simulink model "VSDk_PMSM_6"  (R2024a)
settings: Solver=VariableStepAuto  StartTime=0.0  StopTime=10.0  RelTol=1e-3
values from neighbouring files (symbols this model uses):
  faif = 0.1351    [init.m]
  Iq_limit = Tn/(1.5*p*faif)*1    (= 90.6192943499)    [init.m]
  Jm = 0.36    [init.m]
  Ki_id_vsd = Rs * wc    (= 61.7197292724)    [init.m]
  Ki_iq_vsd = Rs * wc    (= 61.7197292724)    [init.m]
  Ki_x = Rs * wc_xy    (= 61.7197292724)    [init.m]
  Ki_y = Rs * wc_xy    (= 61.7197292724)    [init.m]
  Kis_vsd = (ws^2 * Jm) / KT    (= 438.324399752)    [init.m]
  Kp_id_vsd = Ld_eff * wc    (= 0.485061905714)    [init.m]
  Kp_iq_vsd = Lq_eff * wc    (= 0.485061905714)    [init.m]
  Kp_x = Lx * wc_xy    (= 0.020106192983)    [init.m]
  Kp_y = Ly * wc_xy    (= 0.020106192983)    [init.m]
  Kps_vsd = (2 * zeta * ws * Jm) / KT    (= 19.7285507573)    [init.m]
  LD = Ld+Ldd    (= 7.72e-05)    [init.m]
  Ld = 40.2e-6    (= 4.02e-05)    [init.m]
  Ldd = 37e-6    (= 3.7e-05)    [init.m]
  Ldz = Ld-Ldd    (= 3.2e-06)    [init.m]
  LQ = Lq+Lqq    (= 7.72e-05)    [init.m]
  Lq = 40.2e-6    (= 4.02e-05)    [init.m]
  Lqq = 37e-6    (= 3.7e-05)    [init.m]
  n = 2000    [init.m]
  p = 4    [init.m]
  Rs = 9.823e-3    (= 0.009823)    [init.m]
  Tn = 734.56/10    (= 73.456)    [init.m]
  Ts = 1/(16e3)    (= 6.25e-05)    [init.m]
  Ts_FEA = 1e-7    (= 1e-07)    [init.m]
  VDC = 1200    [init.m]
  wc_xy = 2 * pi * fc_xy    (= 6283.18530718)    [init.m]
libraries: spsIGBTDiodeLib x24, spsVoltageMeasurementLib x16, spsSeriesRLCBranchLib x12, spsDiodeLib x12, spsOnDelayLib x12, slpidlib x11, simulink x7, spsControlledCurrentSourceLib x6, spsDCVoltageSourceLib x1, spsdq0toAlphaBetaZeroLib x1, spspowerguiLib x1
(part 1 of 3)
settings Model: SimulationMode=accelerator  Creator=Downstream  LastModifiedBy=NitrenePL-SAT
settings DebuggingCC: UnderspecifiedInitializationDetection=Classic  MergeDetectMultiDrivingBlocksExec=none
settings ModelReferenceCC: PropagateSignalLabelsOutOfModel=off

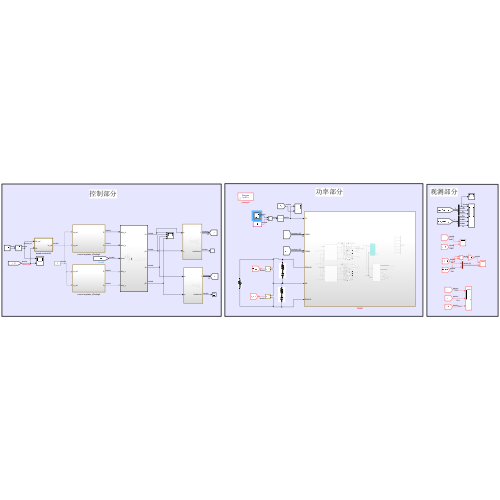
[thumbnail: Simulink's stored preview of the top-level diagram]
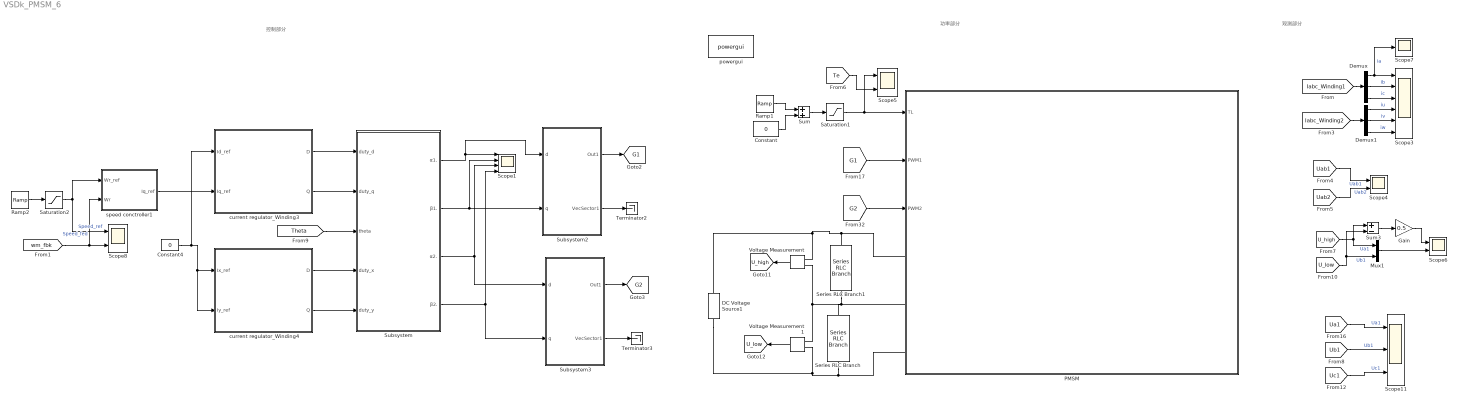
== system VSDk_PMSM_6 ==
  note: 功率部分
  note: 观测部分
  note: 控制部分
  Constant : Constant  Value=0
  Constant4 : Constant  Value=0  SampleTime=-1
  DC Voltage Source1 : spsDCVoltageSourceLib/DC Voltage Source  Amplitude=VDC  Measurements=None
  Demux : Demux  Outputs=3
  Demux1 : Demux  Outputs=3
  Gain : Gain  Gain=0.5
  Mux1 : Mux  Inputs=2
  PMSM : Subsystem
  Ramp1 : simulink/Sources/Ramp  slope=Tn  start=3  InitialOutput=0
  Ramp2 : simulink/Sources/Ramp  slope=n  start=0  InitialOutput=0
  Saturation1 : Saturate  UpperLimit=Tn
  Saturation2 : Saturate  UpperLimit=n
  Scope1 : Scope  NumInputPorts=4
  Scope11 : Scope  NumInputPorts=3
  Scope3 : Scope  NumInputPorts=6
  Scope{4..6,8} (4 alike) : Scope  NumInputPorts=2
  Scope7 : Scope
  Series RLC Branch : spsSeriesRLCBranchLib/Series RLC Branch  LConnTagsString=__new0  RConnTagsString=__new0  BranchType=RC  Resistance=1e-3  Inductance=0  SetiL0=off  InitialCurrent=0  Capacitance=1000e-6  Setx0=off  InitialVoltage=0  Measurements=None
  Series RLC Branch1 : spsSeriesRLCBranchLib/Series RLC Branch  LConnTagsString=__new0  RConnTagsString=__new0  BranchType=RC  Resistance=1e-3  Inductance=0  SetiL0=off  InitialCurrent=0  Capacitance=1000e-6  Setx0=off  InitialVoltage=0  Measurements=None
  Subsystem : Subsystem
  Subsystem2 : Subsystem
  Subsystem3 : Subsystem
  Sum : Sum  OutMax=[Tn]
  Sum3 : Sum  Inputs=+-
  Terminator2 : Terminator
  Terminator3 : Terminator
  Voltage Measurement : spsVoltageMeasurementLib/Voltage Measurement  PhasorSimulation=off  OutputType=Complex  PSBequivalent=0
  Voltage Measurement1 : spsVoltageMeasurementLib/Voltage Measurement  PhasorSimulation=off  OutputType=Complex  PSBequivalent=0
  current regulator_Winding3 : Subsystem
  current regulator_Winding4 : Subsystem
  powergui : spspowerguiLib/powergui  Priority=1  SimulationMode=Discrete  SampleTime=Ts_FEA  frequency=60  Iterations=50  frequencyindice=0  Pbase=100e6  ErrMax=1e-4  UnitsV=kV  UnitsW=MW  buscounter=0  FunctionMessages=off  echomessages=off  EnableUseOfTLC=off  CurrentSourceSwitches=off  DisableSnubberDevices=off  DisableRonSwitches=off  DisableVfSwitches=off  DisplayEquations=off  AutomaticDiscreteSolvers=off  SolverType=Tustin/Backward Euler (TBE)  Interpol=off  ExternalGateDelay=off  methode=off  Ts=100  x0status=blocks  SPID=on  SwTol=0  HookPort=off  NonlinearTolerance=1e-4  nMaxIteration=100  ContinueOnMaxIteration=off  RestoreLinks=warning  ResistiveCurrentMeasurement=off  Frange=[0:2:500]  Ylog=off  Xlog=on  ShowGrid=off  save=off  variable=ZData  structure=IA  ZoomFFT=on  StartTime=0.1927030  cycles=3  DisplayStyle=2  fundamental=816.67  FreqAxis=on  MaxFrequency=816.67*10  frequencyindicesteady=1  RmsSteady=1  display=off
  speed conctroller1 : Subsystem  TreatAsAtomicUnit=on
  tag scope: G1=global, G2=global, U_high=global, U_low=global
  wires:
  [G2] -> PMSM/3(PWM2)
  [G1] -> PMSM/2(PWM1)
  Voltage Measurement1/1 -> [U_low]
  Voltage Measurement/1 -> [U_high]
  Ramp1/1 -> Sum/1
  Constant/1 -> Sum/2
  [Iabc_Winding1] -> Demux/1
  [Iabc_Winding2] -> Demux1/1
  Demux1/3 -> Scope3/6  "iw"
  Demux1/2 -> Scope3/5  "iv"
  Demux1/1 -> Scope3/4  "iu"
  Demux/3 -> Scope3/3  "ic"
  Demux/2 -> Scope3/2  "ib"
  Demux/1 -> Scope7/1, Scope3/1  "ia"
  [Uab1] -> Scope4/1  "Uab1"
  [Uab2] -> Scope4/2  "Uab2"
  Sum/1 -> Saturation1/1
  Saturation1/1 -> PMSM/1(TL), Scope5/1
  [Te] -> Scope5/2
  Constant4/1 -> current regulator_Winding3/1(Id_ref), current regulator_Winding4/2(Iy_ref), current regulator_Winding4/1(Ix_ref)
  Subsystem2/2(VecSector1) -> Terminator2/1
  Subsystem2/1(Out1) -> [G1]
  Ramp2/1 -> Saturation2/1
  Subsystem3/2(VecSector1) -> Terminator3/1
  Saturation2/1 -> speed conctroller1/1(Wr_ref), Scope8/1  "Speed_ref"
  Subsystem3/1(Out1) -> [G2]
  speed conctroller1/1(Iq_ref) -> current regulator_Winding3/2(Iq_ref)
  [Ua1] -> Scope11/1  "Ua1"
  [Ub1] -> Scope11/2  "Ub1"
  [Uc1] -> Scope11/3  "Uc1"
  Sum3/1 -> Gain/1
  [U_high] -> Mux1/1, Sum3/1  "Ua1"
  [U_low] -> Mux1/2, Sum3/2  "Ub1"
  Gain/1 -> Scope6/1
  Mux1/1 -> Scope6/2
  [Theta] -> Subsystem/3(theta)
  current regulator_Winding3/1(D) -> Subsystem/1(duty_d)
  current regulator_Winding3/2(Q) -> Subsystem/2(duty_q)
  current regulator_Winding4/1(D) -> Subsystem/4(duty_x)
  current regulator_Winding4/2(Q) -> Subsystem/5(duty_y)
  Subsystem/1(α1.) -> Subsystem2/1(d), Scope1/1
  Subsystem/4(β2.) -> Subsystem3/2(q), Scope1/4
  Subsystem/2(β1.) -> Subsystem2/2(q), Scope1/2
  Subsystem/3(α2.) -> Scope1/3, Subsystem3/1(d)
  [wm_fbk] -> Scope8/2, speed conctroller1/2(Wr)  "Speed_fed"
  connections:
  Voltage Measurement1/LConn2 -- DC Voltage Source1/LConn1 -- PMSM/LConn3 -- Series RLC Branch/RConn1
  Voltage Measurement/LConn1 -- DC Voltage Source1/RConn1 -- Series RLC Branch1/LConn1 -- PMSM/LConn1
  Voltage Measurement/LConn2 -- Series RLC Branch/LConn1 -- Series RLC Branch1/RConn1 -- PMSM/LConn2 -- Voltage Measurement1/LConn1

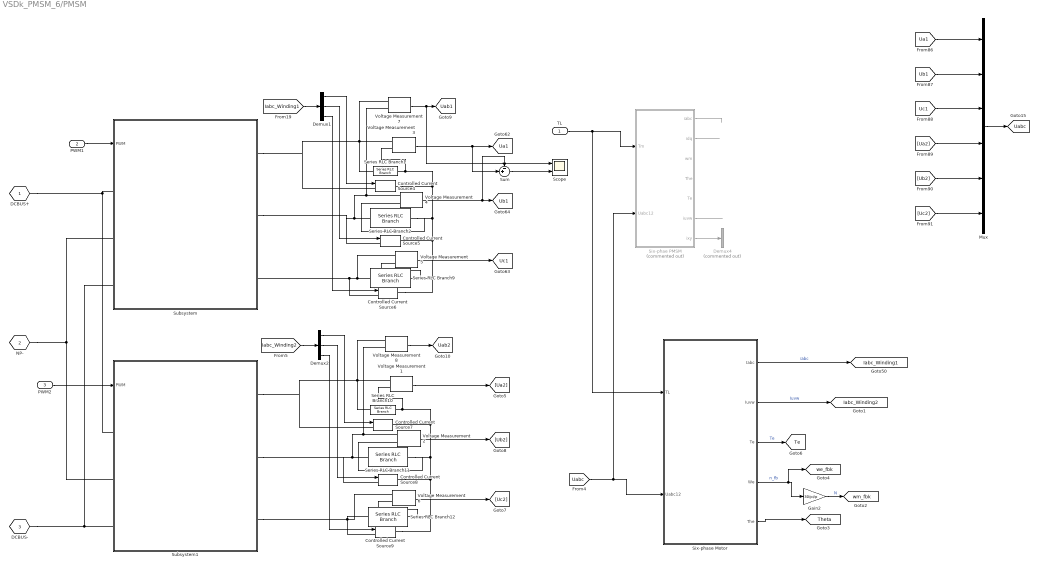
== system VSDk_PMSM_6/PMSM ==
  TL : Inport
  PWM1 : Inport  Port=2
  PWM2 : Inport  Port=3
  Controlled Current Source{4..9} (6 alike) : spsControlledCurrentSourceLib/Controlled Current Source  Initialize=on  Source_Type=AC  Amplitude=0  Phase=0  Frequency=0  Measurements=None
  Demux1 : Demux  Outputs=3
  Demux2 : Demux  Outputs=3
  Demux4 : Demux  Commented=on  Outputs=2
  Gain2 : Gain  Gain=30/pi/p
  Mux : Mux  Inputs=6
  Scope : Scope  NumInputPorts=2
  Series RLC Branch{1..2,9..12} (6 alike) : spsSeriesRLCBranchLib/Series RLC Branch  LConnTagsString=__new0  RConnTagsString=__new0  BranchType=R  Resistance=10^6  Inductance=1e-3  SetiL0=off  InitialCurrent=0  Capacitance=1e-6  Setx0=off  InitialVoltage=0  Measurements=None
  Six-phae PMSM : Subsystem  Commented=on  mask{R=Rs, Ld=LD, Lq=LQ, Lz=Ldz, Flux=faif, J=Jm, F=0, p=p}
      mask prompts: R "R(ohm)"; Ld "Ld(H)"; Lq "Lq(H)"; Lz "Lz(H)"; Flux "Flux(Wb)"; J "J(kg.m^2)"; F "F(N.m.s)"
  Six-phase Motor : Subsystem  mask{Rs=Rs, Ld=Ld, Lq=Lq, Ldd=Ldd, Lqq=Lqq, Flux=faif, B=0, Pn=p, J=Jm}
      mask prompts: Rs "R(ohm)"; Ld "Ld(H)"; Lq "Lq(H)"; Ldd "Ldd(H)"; Lqq "Lqq(H)"; Flux "Flux(wb)"; J "J(kg*m^2)"
      mask DialogControl DescTextVar Prompt: six phase motor
      mask DialogControl Control2 Prompt: Stator Resistance
      mask DialogControl Rs Tooltip: Stator Resistance
      mask DialogControl Control3 Prompt: Stator  d axis Inductance
      mask DialogControl Control4 Prompt: Stator  q axis Inductance
      mask DialogControl Control5 Prompt: Stator  d axis Mutual Inductance
      mask DialogControl Control6 Prompt: Stator  q axis Mutual Inductance
      mask DialogControl Control7 Prompt: Flux linkage
      mask DialogControl Control8 Prompt: damping coefficient
      mask DialogControl Control9 Prompt: motor pole pairs
      mask DialogControl Control10 Prompt: rotational intertia
  Subsystem : Subsystem
  Subsystem1 : Subsystem
  Sum : Sum  Inputs=-+|
  Voltage Measurement{1..8} (8 alike) : spsVoltageMeasurementLib/Voltage Measurement  PhasorSimulation=off  OutputType=Complex  PSBequivalent=0
  DCBUS+ : PMIOPort  Tag=PMCPort  Side=Left
  NP- : PMIOPort  Tag=PMCPort  Port=2  Side=Left
  DCBUS- : PMIOPort  Tag=PMCPort  Port=3  Side=Left
  tag scope: Iabc_Winding1=global, Iabc_Winding2=global, Te=global, Theta=global, Ua1=global, Uab1=global, Uab2=global, Uabc=global, Ub1=global, Uc1=global, we_fbk=global, wm_fbk=global
  wires:
  [Uc2] -> Mux/6
  [Ua2] -> Mux/4
  [Ua1] -> Mux/1
  [Ub1] -> Mux/2
  [Ub2] -> Mux/5
  [Uc1] -> Mux/3
  Mux/1 -> [Uabc]
  Six-phase Motor/4(We) -> Gain2/1, [we_fbk]  "n_fb"
  Six-phase Motor/5(The) -> [Theta]
  Six-phase Motor/3(Te) -> [Te]  "Te"
  PWM1/1 -> Subsystem/1(PWM)
  PWM2/1 -> Subsystem1/1(PWM)
  Demux1/3 -> Controlled Current Source6/1
  Voltage Measurement3/1 -> Sum/2, [Ua1]
  Demux1/2 -> Controlled Current Source5/1
  Voltage Measurement5/1 -> [Uc1]
  Demux1/1 -> Controlled Current Source4/1
  [Iabc_Winding1] -> Demux1/1
  Demux2/2 -> Controlled Current Source8/1
  [Iabc_Winding2] -> Demux2/1
  Demux2/3 -> Controlled Current Source9/1
  Voltage Measurement1/1 -> [Ua2]
  Demux2/1 -> Controlled Current Source7/1
  Voltage Measurement2/1 -> [Ub2]
  Voltage Measurement6/1 -> [Uc2]
  Voltage Measurement7/1 -> Scope/1, [Uab1]
  Voltage Measurement8/1 -> [Uab2]
  TL/1 -> Six-phase Motor/1(TL), Six-phae PMSM/1(Tm)
  Gain2/1 -> [wm_fbk]  "N"
  Six-phae PMSM/7(ixy) -> Demux4/1
  Voltage Measurement4/1 -> Sum/1, [Ub1]
  Sum/1 -> Scope/2
  Six-phase Motor/1(Iabc) -> [Iabc_Winding1]  "iabc"
  Six-phase Motor/2(Iuvw) -> [Iabc_Winding2]  "Iuvw"
  Six-phae PMSM/1(iabc) -> ?
  Six-phae PMSM/2(idq) -> ?
  Six-phae PMSM/6(iuvw) -> ?
  [Uabc] -> Six-phae PMSM/2(Uabc12), Six-phase Motor/2(Uabc12)
  connections:
  DCBUS+/RConn1 -- Subsystem1/LConn1 -- Subsystem/LConn1
  NP-/RConn1 -- Subsystem/LConn2 -- Subsystem1/LConn2
  DCBUS-/RConn1 -- Subsystem1/LConn3 -- Subsystem/LConn3
  Voltage Measurement3/LConn2 -- Series RLC Branch1/LConn1 -- Controlled Current Source4/RConn1 -- Voltage Measurement4/LConn2 -- Series RLC Branch2/LConn1 -- Controlled Current Source5/RConn1 -- Controlled Current Source6/RConn1 -- Series RLC Branch9/LConn1 -- Voltage Measurement5/LConn2
  Voltage Measurement5/LConn1 -- Series RLC Branch9/RConn1 -- Controlled Current Source6/LConn1 -- Subsystem/RConn3
  Voltage Measurement4/LConn1 -- Voltage Measurement7/LConn2 -- Series RLC Branch2/RConn1 -- Subsystem/RConn2 -- Controlled Current Source5/LConn1
  Voltage Measurement3/LConn1 -- Series RLC Branch1/RConn1 -- Voltage Measurement7/LConn1 -- Controlled Current Source4/LConn1 -- Subsystem/RConn1
  Controlled Current Source9/LConn1 -- Subsystem1/RConn3 -- Series RLC Branch12/RConn1 -- Voltage Measurement6/LConn1
  Voltage Measurement1/LConn2 -- Series RLC Branch10/LConn1 -- Controlled Current Source7/RConn1 -- Voltage Measurement2/LConn2 -- Series RLC Branch11/LConn1 -- Controlled Current Source8/RConn1 -- Controlled Current Source9/RConn1 -- Series RLC Branch12/LConn1 -- Voltage Measurement6/LConn2
  Voltage Measurement2/LConn1 -- Voltage Measurement8/LConn2 -- Series RLC Branch11/RConn1 -- Subsystem1/RConn2 -- Controlled Current Source8/LConn1
  Voltage Measurement1/LConn1 -- Voltage Measurement8/LConn1 -- Subsystem1/RConn1 -- Controlled Current Source7/LConn1 -- Series RLC Branch10/RConn1

== system VSDk_PMSM_6/Subsystem ==
  duty_d : Inport
  duty_q : Inport  Port=2
  theta : Inport  Port=3
  duty_x : Inport  Port=4
  duty_y : Inport  Port=5
  Constant2 : Constant  Value=0
  Demux2 : Demux  Outputs=3
  Mux : Mux  Inputs=3
  Mux2 : Mux
  Scope : Scope
  dq0 to Alpha-Beta-Zero : spsdq0toAlphaBetaZeroLib/dq0 to Alpha-Beta-Zero  Alignment=Aligned with phase A axis
  α1 : Fcn  Expr=u(1)+u(3)
  α2 : Fcn  Expr=(sqrt(3)*u(1)+u(2)-sqrt(3)*u(3)+u(4))/2
  β1 : Fcn  Expr=u(2)-u(4)
  β2 : Fcn  Expr=(-u(1)+sqrt(3)*u(2)+u(3)+sqrt(3)*u(4))/2
  α1. : Outport
  β1. : Outport  Port=2
  α2. : Outport  Port=3
  β2. : Outport  Port=4
  wires:
  duty_x/1 -> Mux2/3
  Demux2/1 -> Mux2/1
  Mux/1 -> dq0 to Alpha-Beta-Zero/1
  Constant2/1 -> Mux/3
  Mux2/1 -> Scope/1, β2/1, α2/1, α1/1, β1/1
  duty_y/1 -> Mux2/4
  Demux2/2 -> Mux2/2
  dq0 to Alpha-Beta-Zero/1 -> Demux2/1
  duty_q/1 -> Mux/2
  duty_d/1 -> Mux/1
  theta/1 -> dq0 to Alpha-Beta-Zero/2
  α1/1 -> α1./1
  β1/1 -> β1./1
  α2/1 -> α2./1
  β2/1 -> β2./1

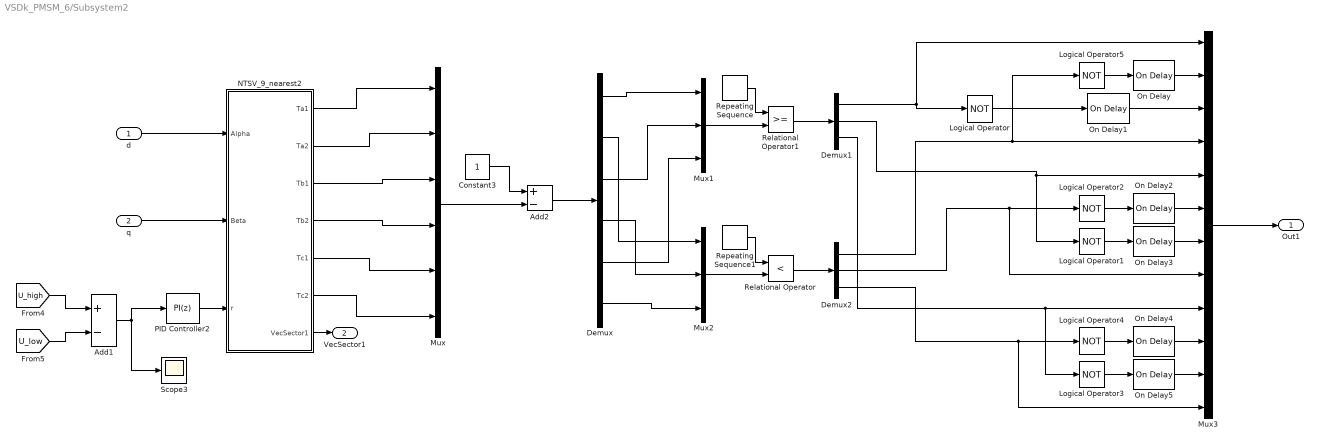
== system VSDk_PMSM_6/Subsystem2 ==
  d : Inport
  q : Inport  Port=2
  Add1 : Sum  Inputs=+-
  Add2 : Sum  Inputs=+-
  Constant3 : Constant
  Demux : Demux  Outputs=6
  Demux1 : Demux  Outputs=3
  Demux2 : Demux  Outputs=3
  Logical Operator{,1..5} (6 alike) : Logic  Operator=NOT  AllPortsSameDT=off  OutDataTypeStr=boolean
  Mux : Mux  Inputs=6
  Mux1 : Mux  Inputs=3
  Mux2 : Mux  Inputs=3
  Mux3 : Mux  Inputs=12
  NTSV_9_nearest2 : MATLAB Function  TreatAsAtomicUnit=on
  On Delay{,1..5} (6 alike) : spsOnDelayLib/On Delay  DelayType=On delay  delay=Ts_Dead  ic=0  Ts=0
  PID Controller2 : slpidlib/PID Controller  Controller=PI  Form=Parallel  TimeDomain=Discrete-time  UseExternalTs=off  SampleTime=Ts  IntegratorMethod=Forward Euler  FilterMethod=Forward Euler  ControllerParametersSource=internal  P=0.005  I=0.05  UseKiTs=off  D=0  UseExternalDerivativeSource=off  N=100  UseFilter=on  TunerSelectOption=Transfer Function Based (PID Tuner App)  InitialConditionSource=internal  InitialConditionForIntegrator=0  InitialConditionForFilter=0  DifferentiatorICPrevScaledInput=0  ExternalReset=none  TrackingMode=off  Kt=1  LimitOutput=off  SatLimitsSource=internal  UpperSaturationLimit=inf  LowerSaturationLimit=-inf  LinearizeAsGain=on  AntiWindupMode=none  Kb=1  LimitIntegrator=off  UpperIntegratorSaturationLimit=inf  LowerIntegratorSaturationLimit=-inf  POutMin=[]  POutMax=[]  IOutMin=[]  IOutMax=[]  DOutMin=[]  DOutMax=[]  NOutMin=[]  NOutMax=[]  SumOutMin=[]  SumOutMax=[]  SaturationOutMin=[]  SaturationOutMax=[]  PParamMin=[]  PParamMax=[]  IParamMin=[]  IParamMax=[]  DParamMin=[]  DParamMax=[]  NParamMin=[]  NParamMax=[]  KbParamMin=[]  KbParamMax=[]  KtParamMin=[]  KtParamMax=[]  KbOutMin=[]  KbOutMax=[]  KtOutMin=[]  KtOutMax=[]  IntegratorOutMin=[]  IntegratorOutMax=[]  FilterOutMin=[]  FilterOutMax=[]  SumI1OutMin=[]  SumI1OutMax=[]  SumI2OutMin=[]  SumI2OutMax=[]  SumI3OutMin=[]  SumI3OutMax=[]  SumI4OutMin=[]  SumI4OutMax=[]  SumDOutMin=[]  SumDOutMax=[]  DifferentiatorOutMin=[]  DifferentiatorOutMax=[]  FilterDiffOutCoefMin=[]  FilterDiffOutCoefMax=[]  ReciprocalOutMin=[]  ReciprocalOutMax=[]  SumDenOutMin=[]  SumDenOutMax=[]  SumNumOutMin=[]  SumNumOutMax=[]  DivideOutMin=[]  DivideOutMax=[]  UdiffTsProdOutMin=[]  UdiffTsProdOutMax=[]  NTsProdOutMin=[]  NTsProdOutMax=[]  UintegralTsProdOutMin=[]  UintegralTsProdOutMax=[]  UngainTsProdOutMin=[]  UngainTsProdOutMax=[]  ClampingZeroOutDataTypeStr=Inherit: Inherit via back propagation  ClampingZeroOutMin=[]  ClampingZeroOutMax=[]  FilterDenConstantOutDataTypeStr=Inherit: Inherit via back propagation  FilterDenConstantOutMin=[]  FilterDenConstantOutMax=[]  PCopyOutDataTypeStr=Inherit: Inherit via back propagation  PCopyOutMin=[]  PCopyOutMax=[]  NCopyOutDataTypeStr=Inherit: Inherit via back propagation  NCopyOutMin=[]  NCopyOutMax=[]  IntegratorContinuousStateAttributes=''  IntegratorStateMustResolveToSignalObject=off  IntegratorRTWStateStorageClass=Auto  FilterContinuousStateAttributes=''  FilterStateMustResolveToSignalObject=off  FilterRTWStateStorageClass=Auto  ParallelPVariant=InternalParameters  IdealPVariant=Disabled  IVariant=InternalParameters  DVariant=Disabled  IntegratorVariant=Discrete  SatVariant=Disabled  AWVariant=Passthrough  PCopyVariant=Disabled  TRVariant=Disabled  FdbkBlocksVariant=Forward  IdealPFdbkVariant=Disabled  SatFdbkVariant=Disabled  DerivativeFilterVariant=Disabled  NVariant=Disabled  NCopyVariant=Disabled_SignalSpec  FilterICVariant=Disabled  IntegratorICVariant=InternalICs  ExternalResetVariant=Disabled  TRSumVariant=Passthrough  SumFdbkVariant=Disabled  SumVariant=Sum_PI  TsampFilterVariant=InternalTs  TsampNgainVariant=Passthrough  TsampIntegralVariant=Disabled_SignalSpec  ExternalSaturationOutDataTypeStr=Inherit: Same as second input  DerivativeSourceVariant=Disabled
  Relational Operator : RelationalOperator  Operator=<  OutDataTypeStr=boolean  RndMeth=Simplest  InputSameDT=off
  Relational Operator1 : RelationalOperator  OutDataTypeStr=boolean  RndMeth=Simplest  InputSameDT=off
  Repeating Sequence : simulink/Sources/Repeating Sequence  rep_seq_t=[0 Ts/2 Ts]  rep_seq_y=[0 1 0]
  Repeating Sequence1 : simulink/Sources/Repeating Sequence  rep_seq_t=[0 Ts/2 Ts]  rep_seq_y=[0 1 0]
  Scope3 : Scope
  Out1 : Outport
  VecSector1 : Outport  Port=2
  wires:
  NTSV_9_nearest2/7(VecSector1) -> VecSector1/1
  Demux/1 -> Mux1/1
  Demux2/3 -> Logical Operator4/1, Mux3/12
  Logical Operator4/1 -> On Delay4/1
  Demux/5 -> Mux1/3
  Logical Operator2/1 -> On Delay2/1
  Demux1/1 -> Logical Operator/1, Mux3/1
  Add1/1 -> Scope3/1, PID Controller2/1
  Constant3/1 -> Add2/1
  Demux2/2 -> Mux3/8, Logical Operator2/1
  Demux2/1 -> Logical Operator5/1, Mux3/4
  On Delay1/1 -> Mux3/3
  NTSV_9_nearest2/2(Ta2) -> Mux/2
  On Delay3/1 -> Mux3/7
  Logical Operator5/1 -> On Delay/1
  Relational Operator1/1 -> Demux1/1
  Mux/1 -> Add2/2
  Repeating Sequence1/1 -> Relational Operator/1
  NTSV_9_nearest2/6(Tc2) -> Mux/6
  Demux/2 -> Mux2/1
  Mux1/1 -> Relational Operator1/2
  Mux2/1 -> Relational Operator/2
  PID Controller2/1 -> NTSV_9_nearest2/3(r)
  Add2/1 -> Demux/1
  On Delay/1 -> Mux3/2
  Relational Operator/1 -> Demux2/1
  NTSV_9_nearest2/1(Ta1) -> Mux/1
  [U_low] -> Add1/2
  NTSV_9_nearest2/4(Tb2) -> Mux/4
  Demux/6 -> Mux2/3
  Demux1/3 -> Logical Operator3/1, Mux3/9
  q/1 -> NTSV_9_nearest2/2(Beta)
  On Delay2/1 -> Mux3/6
  [U_high] -> Add1/1
  On Delay5/1 -> Mux3/11
  NTSV_9_nearest2/5(Tc1) -> Mux/5
  Demux1/2 -> Logical Operator1/1, Mux3/5
  d/1 -> NTSV_9_nearest2/1(Alpha)
  Logical Operator3/1 -> On Delay5/1
  On Delay4/1 -> Mux3/10
  Mux3/1 -> Out1/1
  NTSV_9_nearest2/3(Tb1) -> Mux/3
  Logical Operator/1 -> On Delay1/1
  Logical Operator1/1 -> On Delay3/1
  Repeating Sequence/1 -> Relational Operator1/1
  Demux/4 -> Mux2/2
  Demux/3 -> Mux1/2

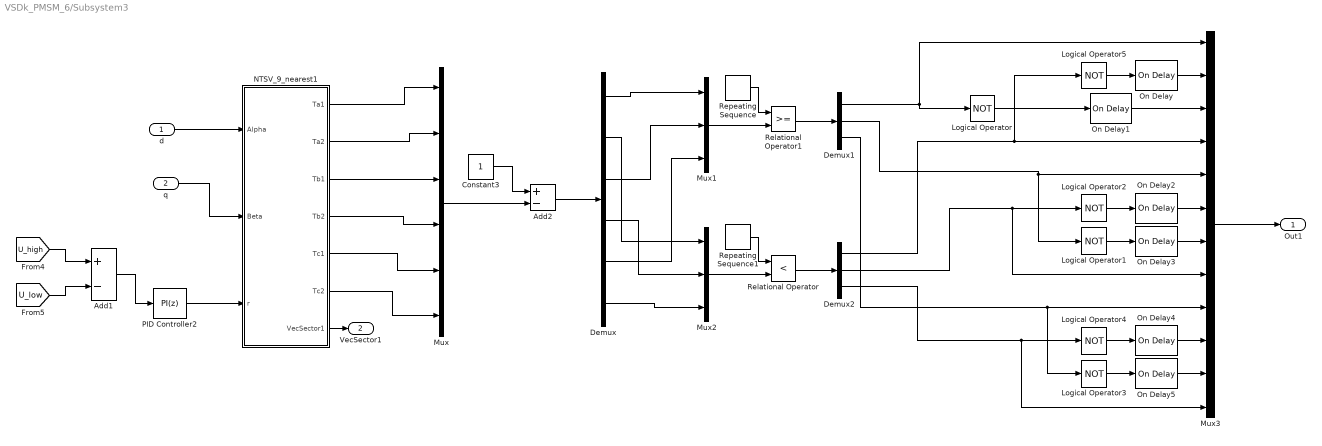
== system VSDk_PMSM_6/Subsystem3 ==
  d : Inport
  q : Inport  Port=2
  Add1 : Sum  Inputs=+-
  Add2 : Sum  Inputs=+-
  Constant3 : Constant
  Demux : Demux  Outputs=6
  Demux1 : Demux  Outputs=3
  Demux2 : Demux  Outputs=3
  Logical Operator{,1..5} (6 alike) : Logic  Operator=NOT  AllPortsSameDT=off  OutDataTypeStr=boolean
  Mux : Mux  Inputs=6
  Mux1 : Mux  Inputs=3
  Mux2 : Mux  Inputs=3
  Mux3 : Mux  Inputs=12
  NTSV_9_nearest1 : MATLAB Function  TreatAsAtomicUnit=on
  On Delay{,1..5} (6 alike) : spsOnDelayLib/On Delay  DelayType=On delay  delay=Ts_Dead  ic=0  Ts=0
  PID Controller2 : slpidlib/PID Controller  Controller=PI  Form=Parallel  TimeDomain=Discrete-time  UseExternalTs=off  SampleTime=Ts  IntegratorMethod=Forward Euler  FilterMethod=Forward Euler  ControllerParametersSource=internal  P=0.005  I=0.05  UseKiTs=off  D=0  UseExternalDerivativeSource=off  N=100  UseFilter=on  TunerSelectOption=Transfer Function Based (PID Tuner App)  InitialConditionSource=internal  InitialConditionForIntegrator=0  InitialConditionForFilter=0  DifferentiatorICPrevScaledInput=0  ExternalReset=none  TrackingMode=off  Kt=1  LimitOutput=off  SatLimitsSource=internal  UpperSaturationLimit=inf  LowerSaturationLimit=-inf  LinearizeAsGain=on  AntiWindupMode=none  Kb=1  LimitIntegrator=off  UpperIntegratorSaturationLimit=inf  LowerIntegratorSaturationLimit=-inf  POutMin=[]  POutMax=[]  IOutMin=[]  IOutMax=[]  DOutMin=[]  DOutMax=[]  NOutMin=[]  NOutMax=[]  SumOutMin=[]  SumOutMax=[]  SaturationOutMin=[]  SaturationOutMax=[]  PParamMin=[]  PParamMax=[]  IParamMin=[]  IParamMax=[]  DParamMin=[]  DParamMax=[]  NParamMin=[]  NParamMax=[]  KbParamMin=[]  KbParamMax=[]  KtParamMin=[]  KtParamMax=[]  KbOutMin=[]  KbOutMax=[]  KtOutMin=[]  KtOutMax=[]  IntegratorOutMin=[]  IntegratorOutMax=[]  FilterOutMin=[]  FilterOutMax=[]  SumI1OutMin=[]  SumI1OutMax=[]  SumI2OutMin=[]  SumI2OutMax=[]  SumI3OutMin=[]  SumI3OutMax=[]  SumI4OutMin=[]  SumI4OutMax=[]  SumDOutMin=[]  SumDOutMax=[]  DifferentiatorOutMin=[]  DifferentiatorOutMax=[]  FilterDiffOutCoefMin=[]  FilterDiffOutCoefMax=[]  ReciprocalOutMin=[]  ReciprocalOutMax=[]  SumDenOutMin=[]  SumDenOutMax=[]  SumNumOutMin=[]  SumNumOutMax=[]  DivideOutMin=[]  DivideOutMax=[]  UdiffTsProdOutMin=[]  UdiffTsProdOutMax=[]  NTsProdOutMin=[]  NTsProdOutMax=[]  UintegralTsProdOutMin=[]  UintegralTsProdOutMax=[]  UngainTsProdOutMin=[]  UngainTsProdOutMax=[]  ClampingZeroOutDataTypeStr=Inherit: Inherit via back propagation  ClampingZeroOutMin=[]  ClampingZeroOutMax=[]  FilterDenConstantOutDataTypeStr=Inherit: Inherit via back propagation  FilterDenConstantOutMin=[]  FilterDenConstantOutMax=[]  PCopyOutDataTypeStr=Inherit: Inherit via back propagation  PCopyOutMin=[]  PCopyOutMax=[]  NCopyOutDataTypeStr=Inherit: Inherit via back propagation  NCopyOutMin=[]  NCopyOutMax=[]  IntegratorContinuousStateAttributes=''  IntegratorStateMustResolveToSignalObject=off  IntegratorRTWStateStorageClass=Auto  FilterContinuousStateAttributes=''  FilterStateMustResolveToSignalObject=off  FilterRTWStateStorageClass=Auto  ParallelPVariant=InternalParameters  IdealPVariant=Disabled  IVariant=InternalParameters  DVariant=Disabled  IntegratorVariant=Discrete  SatVariant=Disabled  AWVariant=Passthrough  PCopyVariant=Disabled  TRVariant=Disabled  FdbkBlocksVariant=Forward  IdealPFdbkVariant=Disabled  SatFdbkVariant=Disabled  DerivativeFilterVariant=Disabled  NVariant=Disabled  NCopyVariant=Disabled_SignalSpec  FilterICVariant=Disabled  IntegratorICVariant=InternalICs  ExternalResetVariant=Disabled  TRSumVariant=Passthrough  SumFdbkVariant=Disabled  SumVariant=Sum_PI  TsampFilterVariant=InternalTs  TsampNgainVariant=Passthrough  TsampIntegralVariant=Disabled_SignalSpec  ExternalSaturationOutDataTypeStr=Inherit: Same as second input  DerivativeSourceVariant=Disabled
  Relational Operator : RelationalOperator  Operator=<  OutDataTypeStr=boolean  RndMeth=Simplest  InputSameDT=off
  Relational Operator1 : RelationalOperator  OutDataTypeStr=boolean  RndMeth=Simplest  InputSameDT=off
  Repeating Sequence : simulink/Sources/Repeating Sequence  rep_seq_t=[0 Ts/2 Ts]  rep_seq_y=[0 1 0]
  Repeating Sequence1 : simulink/Sources/Repeating Sequence  rep_seq_t=[0 Ts/2 Ts]  rep_seq_y=[0 1 0]
  Out1 : Outport
  VecSector1 : Outport  Port=2
  wires:
  NTSV_9_nearest1/7(VecSector1) -> VecSector1/1
  Demux/1 -> Mux1/1
  Demux2/3 -> Logical Operator4/1, Mux3/12
  Logical Operator4/1 -> On Delay4/1
  Demux/5 -> Mux1/3
  Logical Operator2/1 -> On Delay2/1
  Demux1/1 -> Logical Operator/1, Mux3/1
  Add1/1 -> PID Controller2/1
  Constant3/1 -> Add2/1
  Demux2/2 -> Mux3/8, Logical Operator2/1
  Demux2/1 -> Logical Operator5/1, Mux3/4
  On Delay1/1 -> Mux3/3
  NTSV_9_nearest1/2(Ta2) -> Mux/2
  On Delay3/1 -> Mux3/7
  Logical Operator5/1 -> On Delay/1
  Relational Operator1/1 -> Demux1/1
  Mux/1 -> Add2/2
  Repeating Sequence1/1 -> Relational Operator/1
  NTSV_9_nearest1/6(Tc2) -> Mux/6
  Demux/2 -> Mux2/1
  Mux1/1 -> Relational Operator1/2
  Mux2/1 -> Relational Operator/2
  PID Controller2/1 -> NTSV_9_nearest1/3(r)
  Add2/1 -> Demux/1
  On Delay/1 -> Mux3/2
  Relational Operator/1 -> Demux2/1
  NTSV_9_nearest1/1(Ta1) -> Mux/1
  [U_low] -> Add1/2
  NTSV_9_nearest1/4(Tb2) -> Mux/4
  Demux/6 -> Mux2/3
  Demux1/3 -> Logical Operator3/1, Mux3/9
  q/1 -> NTSV_9_nearest1/2(Beta)
  On Delay2/1 -> Mux3/6
  [U_high] -> Add1/1
  On Delay5/1 -> Mux3/11
  NTSV_9_nearest1/5(Tc1) -> Mux/5
  Demux1/2 -> Logical Operator1/1, Mux3/5
  d/1 -> NTSV_9_nearest1/1(Alpha)
  Logical Operator3/1 -> On Delay5/1
  On Delay4/1 -> Mux3/10
  Mux3/1 -> Out1/1
  NTSV_9_nearest1/3(Tb1) -> Mux/3
  Logical Operator/1 -> On Delay1/1
  Logical Operator1/1 -> On Delay3/1
  Repeating Sequence/1 -> Relational Operator1/1
  Demux/4 -> Mux2/2
  Demux/3 -> Mux1/2

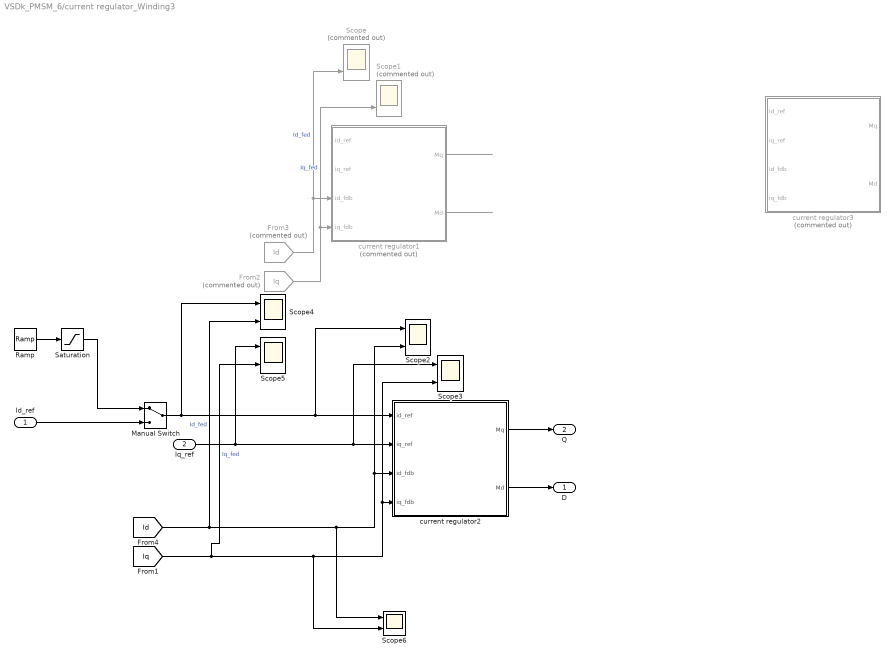
== system VSDk_PMSM_6/current regulator_Winding3 ==
  Id_ref : Inport
  Iq_ref : Inport  Port=2
  From2 : From  Commented=on  GotoTag=Iq  TagVisibility=global
  From3 : From  Commented=on  GotoTag=Id  TagVisibility=global
  Manual Switch : ManualSwitch
  Ramp : simulink/Sources/Ramp  slope=100  start=1.2  InitialOutput=0
  Saturation : Saturate  UpperLimit=200
  Scope : Scope  Commented=on  NumInputPorts=2
  Scope1 : Scope  Commented=on  NumInputPorts=2
  Scope{2..6} (5 alike) : Scope  NumInputPorts=2
  current regulator1 : Subsystem  Commented=on
  current regulator2 : Subsystem
  current regulator3 : Subsystem  Commented=on
  D : Outport  VectorParamsAs1DForOutWhenUnconnected=off
  Q : Outport  Port=2  VectorParamsAs1DForOutWhenUnconnected=off
  wires:
  current regulator1/1(Mq) -> ?
  ? -> Scope/1, current regulator1/1(id_ref)
  current regulator1/2(Md) -> ?
  ? -> Scope1/1, current regulator1/2(iq_ref)
  From3/1 -> Scope/2, current regulator1/3(id_fdb)  "Id_fed"
  From2/1 -> Scope1/2, current regulator1/4(iq_fdb)  "Iq_fed"
  [Iq] -> Scope6/2, Scope3/2, current regulator2/4(iq_fdb), Scope5/2  "Iq_fed"
  [Id] -> Scope6/1, Scope2/2, current regulator2/3(id_fdb), Scope4/2  "Id_fed"
  current regulator2/1(Mq) -> Q/1
  current regulator2/2(Md) -> D/1
  Iq_ref/1 -> Scope3/1, current regulator2/2(iq_ref), Scope5/1
  Ramp/1 -> Saturation/1
  Id_ref/1 -> Manual Switch/2
  Manual Switch/1 -> Scope4/1, Scope2/1, current regulator2/1(id_ref)
  Saturation/1 -> Manual Switch/1

== system VSDk_PMSM_6/current regulator_Winding4 ==
  Ix_ref : Inport
  Iy_ref : Inport  Port=2
  Scope{,1,4..6} (5 alike) : Scope  NumInputPorts=2
  current regulator3 : Subsystem
  D : Outport  VectorParamsAs1DForOutWhenUnconnected=off
  Q : Outport  Port=2  VectorParamsAs1DForOutWhenUnconnected=off
  wires:
  [Iy] -> Scope/2, current regulator3/4(iy_fdb), Scope5/2, Scope6/2  "Iy_fed"
  [Ix] -> Scope/1, current regulator3/3(ix_fdb), Scope4/2, Scope1/2  "Ix_fed"
  Ix_ref/1 -> Scope1/1, current regulator3/1(ix_ref), Scope4/1  "id_fbk"
  Iy_ref/1 -> Scope6/1, current regulator3/2(iy_ref), Scope5/1
  current regulator3/1(My) -> Q/1
  current regulator3/2(Mx) -> D/1

== system VSDk_PMSM_6/speed conctroller1 ==
  Wr_ref : Inport
  Wr : Inport  Port=2
  Add : Sum  Inputs=+-
  PID Controller1 : slpidlib/PID Controller  Controller=PI  Form=Parallel  TimeDomain=Discrete-time  UseExternalTs=off  SampleTime=Ts  IntegratorMethod=Forward Euler  FilterMethod=Forward Euler  ControllerParametersSource=internal  P=Kps_vsd  I=Kis_vsd  UseKiTs=off  D=0  UseExternalDerivativeSource=off  N=100  UseFilter=on  TunerSelectOption=Transfer Function Based (PID Tuner App)  InitialConditionSource=internal  InitialConditionForIntegrator=0  InitialConditionForFilter=0  DifferentiatorICPrevScaledInput=0  ExternalReset=none  TrackingMode=off  Kt=1  LimitOutput=on  SatLimitsSource=internal  UpperSaturationLimit=Iq_limit  LowerSaturationLimit=-Iq_limit  LinearizeAsGain=off  AntiWindupMode=none  Kb=1  LimitIntegrator=off  UpperIntegratorSaturationLimit=inf  LowerIntegratorSaturationLimit=-inf  POutMin=[]  POutMax=[]  IOutMin=[]  IOutMax=[]  DOutMin=[]  DOutMax=[]  NOutMin=[]  NOutMax=[]  SumOutMin=[]  SumOutMax=[]  SaturationOutMin=[]  SaturationOutMax=[]  PParamMin=[]  PParamMax=[]  IParamMin=[]  IParamMax=[]  DParamMin=[]  DParamMax=[]  NParamMin=[]  NParamMax=[]  KbParamMin=[]  KbParamMax=[]  KtParamMin=[]  KtParamMax=[]  KbOutMin=[]  KbOutMax=[]  KtOutMin=[]  KtOutMax=[]  IntegratorOutMin=[]  IntegratorOutMax=[]  FilterOutMin=[]  FilterOutMax=[]  SumI1OutMin=[]  SumI1OutMax=[]  SumI2OutMin=[]  SumI2OutMax=[]  SumI3OutMin=[]  SumI3OutMax=[]  SumI4OutMin=[]  SumI4OutMax=[]  SumDOutMin=[]  SumDOutMax=[]  DifferentiatorOutMin=[]  DifferentiatorOutMax=[]  FilterDiffOutCoefMin=[]  FilterDiffOutCoefMax=[]  ReciprocalOutMin=[]  ReciprocalOutMax=[]  SumDenOutMin=[]  SumDenOutMax=[]  SumNumOutMin=[]  SumNumOutMax=[]  DivideOutMin=[]  DivideOutMax=[]  UdiffTsProdOutMin=[]  UdiffTsProdOutMax=[]  NTsProdOutMin=[]  NTsProdOutMax=[]  UintegralTsProdOutMin=[]  UintegralTsProdOutMax=[]  UngainTsProdOutMin=[]  UngainTsProdOutMax=[]  ClampingZeroOutDataTypeStr=Inherit: Inherit via back propagation  ClampingZeroOutMin=[]  ClampingZeroOutMax=[]  FilterDenConstantOutDataTypeStr=Inherit: Inherit via back propagation  FilterDenConstantOutMin=[]  FilterDenConstantOutMax=[]  PCopyOutDataTypeStr=Inherit: Inherit via back propagation  PCopyOutMin=[]  PCopyOutMax=[]  NCopyOutDataTypeStr=Inherit: Inherit via back propagation  NCopyOutMin=[]  NCopyOutMax=[]  IntegratorContinuousStateAttributes=''  IntegratorStateMustResolveToSignalObject=off  IntegratorRTWStateStorageClass=Auto  FilterContinuousStateAttributes=''  FilterStateMustResolveToSignalObject=off  FilterRTWStateStorageClass=Auto  ParallelPVariant=InternalParameters  IdealPVariant=Disabled  IVariant=InternalParameters  DVariant=Disabled  IntegratorVariant=Discrete  SatVariant=Enabled  AWVariant=Passthrough  PCopyVariant=Disabled  TRVariant=Disabled  FdbkBlocksVariant=Forward  IdealPFdbkVariant=Disabled  SatFdbkVariant=Disabled  DerivativeFilterVariant=Disabled  NVariant=Disabled  NCopyVariant=Disabled_SignalSpec  FilterICVariant=Disabled  IntegratorICVariant=InternalICs  ExternalResetVariant=Disabled  TRSumVariant=Passthrough  SumFdbkVariant=Disabled  SumVariant=Sum_PI  TsampFilterVariant=InternalTs  TsampNgainVariant=Passthrough  TsampIntegralVariant=Disabled_SignalSpec  ExternalSaturationOutDataTypeStr=Inherit: Same as second input  DerivativeSourceVariant=Disabled
  Scope1 : Scope
  Iq_ref : Outport  VectorParamsAs1DForOutWhenUnconnected=off
  wires:
  Add/1 -> PID Controller1/1
  Wr/1 -> Add/2
  PID Controller1/1 -> Iq_ref/1
  Wr_ref/1 -> Scope1/1, Add/1

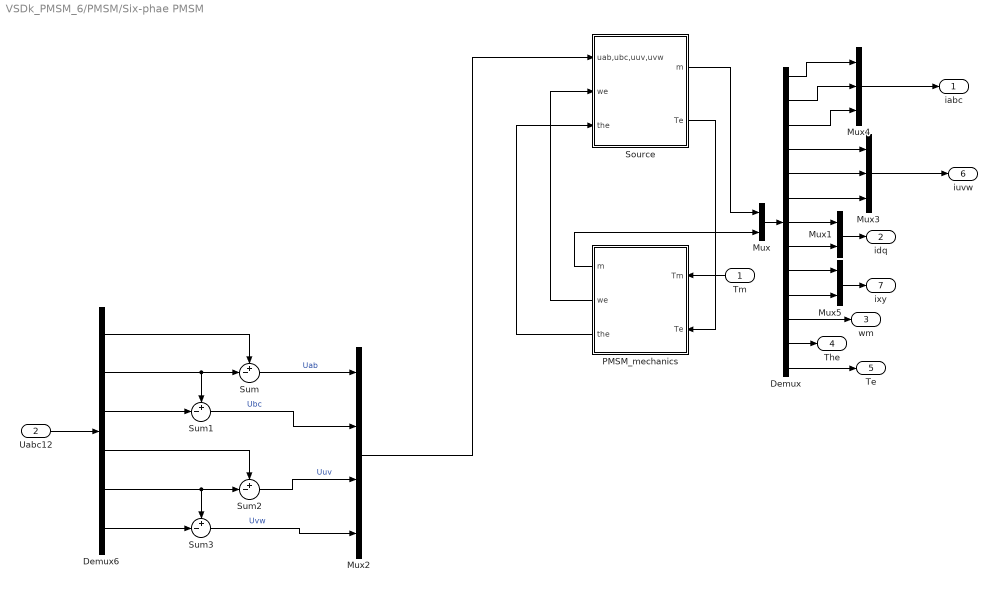
== system VSDk_PMSM_6/PMSM/Six-phae PMSM ==
  Tm : Inport
  Uabc12 : Inport  Port=2
  Demux : Demux  Outputs=13
  Demux6 : Demux  Outputs=6
  Mux : Mux  Inputs=2
  Mux1 : Mux  Inputs=2
  Mux2 : Mux
  Mux3 : Mux  Inputs=3
  Mux4 : Mux  Inputs=3
  Mux5 : Mux  Inputs=2
  PMSM_mechanics : Subsystem
  Source : Subsystem
  Sum{,1..3} (4 alike) : Sum  Inputs=+-|
  iabc : Outport
  idq : Outport  Port=2
  wm : Outport  Port=3
  The : Outport  Port=4
  Te : Outport  Port=5
  iuvw : Outport  Port=6
  ixy : Outport  Port=7
  wires:
  Tm/1 -> PMSM_mechanics/1(Tm)
  Source/2(Te) -> PMSM_mechanics/2(Te)
  PMSM_mechanics/2(we) -> Source/2(we)
  PMSM_mechanics/3(the) -> Source/3(the)
  PMSM_mechanics/1(m) -> Mux/2
  Source/1(m) -> Mux/1
  Mux/1 -> Demux/1
  Mux4/1 -> iabc/1
  Mux1/1 -> idq/1
  Demux/12 -> The/1
  Demux/13 -> Te/1
  Demux/5 -> Mux3/2
  Demux/2 -> Mux4/2
  Demux/3 -> Mux4/3
  Demux/6 -> Mux3/3
  Demux/4 -> Mux3/1
  Demux/1 -> Mux4/1
  Demux/7 -> Mux1/1
  Demux/8 -> Mux1/2
  Demux/9 -> Mux5/1
  Demux/10 -> Mux5/2
  Demux/11 -> wm/1
  Uabc12/1 -> Demux6/1
  Demux6/2 -> Sum1/1, Sum/2
  Demux6/1 -> Sum/1
  Demux6/3 -> Sum1/2
  Sum/1 -> Mux2/1  "Uab"
  Sum1/1 -> Mux2/2  "Ubc"
  Sum3/1 -> Mux2/4  "Uvw"
  Sum2/1 -> Mux2/3  "Uuv"
  Demux6/5 -> Sum3/1, Sum2/2
  Demux6/4 -> Sum2/1
  Demux6/6 -> Sum3/2
  Mux2/1 -> Source/1(uab,ubc,uuv,uvw)
  Mux3/1 -> iuvw/1
  Mux5/1 -> ixy/1

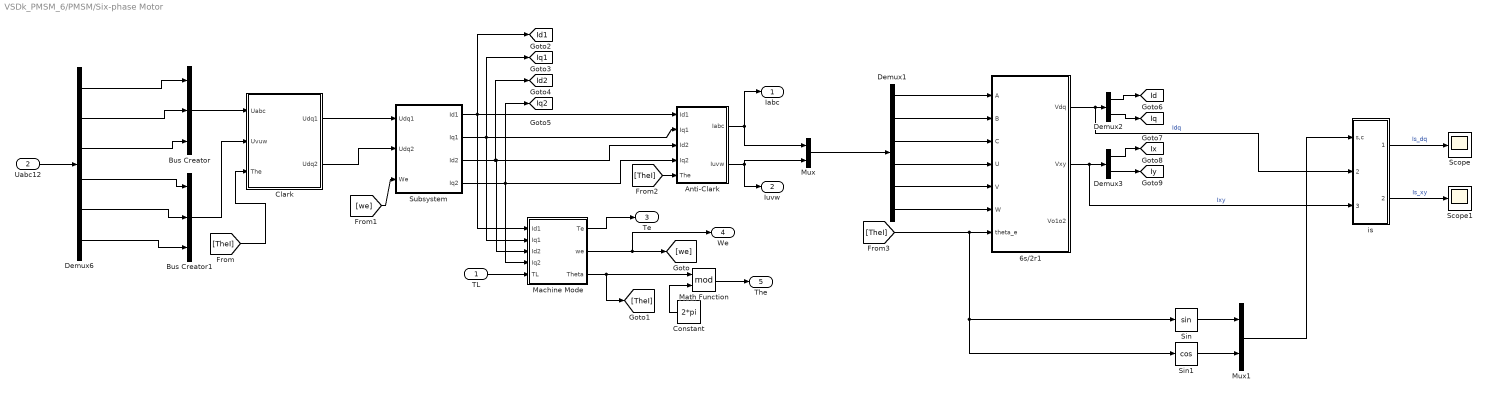
== system VSDk_PMSM_6/PMSM/Six-phase Motor ==
  TL : Inport
  Uabc12 : Inport  Port=2
  6s/2r1 : Subsystem
  Anti-Clark : Subsystem
  Bus Creator : BusCreator  Inputs=3
  Bus Creator1 : BusCreator  Inputs=3
  Clark : Subsystem
  Constant : Constant  Value=2*pi
  Demux1 : Demux  Outputs=6
  Demux2 : Demux  Outputs=2
  Demux3 : Demux  Outputs=2
  Demux6 : Demux  Outputs=6
  Machine Mode : Subsystem
  Math Function : Math  Operator=mod  SignedPower=on
  Mux : Mux  Inputs=2
  Mux1 : Mux  Inputs=2
  Scope : Scope
  Scope1 : Scope
  Sin : Trigonometry
  Sin1 : Trigonometry  Operator=cos
  Subsystem : Subsystem
  is : Subsystem
  Iabc : Outport  VectorParamsAs1DForOutWhenUnconnected=off
  Iuvw : Outport  Port=2  VectorParamsAs1DForOutWhenUnconnected=off
  Te : Outport  Port=3  VectorParamsAs1DForOutWhenUnconnected=off
  We : Outport  Port=4  VectorParamsAs1DForOutWhenUnconnected=off
  The : Outport  Port=5  VectorParamsAs1DForOutWhenUnconnected=off
  tag scope: Id1=global, Id2=global, Id=global, Iq1=global, Iq2=global, Iq=global, Ix=global, Iy=global
  wires:
  Machine Mode/3(Theta) -> Math Function/1, [TheI]
  Anti-Clark/2(Iuvw) -> Mux/2, Iuvw/1
  Anti-Clark/1(Iabc) -> Mux/1, Iabc/1
  [TheI] -> Anti-Clark/5(The)
  Subsystem/4(Iq2) -> [Iq2], Machine Mode/4(Iq2), Anti-Clark/4(Iq2)
  Machine Mode/1(Te) -> Te/1
  [TheI] -> Clark/3(The)
  Machine Mode/2(we) -> [we], We/1
  TL/1 -> Machine Mode/5(TL)
  Subsystem/2(Iq1) -> [Iq1], Machine Mode/2(Iq1), Anti-Clark/2(Iq1)
  Subsystem/1(Id1) -> [Id1], Anti-Clark/1(Id1), Machine Mode/1(Id1)
  Clark/2(Udq2) -> Subsystem/2(Udq2)
  Bus Creator1/1 -> Clark/2(Uvuw)
  Bus Creator/1 -> Clark/1(Uabc)
  Demux6/5 -> Bus Creator1/2
  Demux6/4 -> Bus Creator1/1
  Demux6/6 -> Bus Creator1/3
  Demux6/3 -> Bus Creator/3
  Demux6/2 -> Bus Creator/2
  Demux6/1 -> Bus Creator/1
  Clark/1(Udq1) -> Subsystem/1(Udq1)
  [we] -> Subsystem/3(We)
  Math Function/1 -> The/1
  Constant/1 -> Math Function/2
  Subsystem/3(Id2) -> [Id2], Anti-Clark/3(Id2), Machine Mode/3(Id2)
  Uabc12/1 -> Demux6/1
  Demux2/1 -> [Id]
  6s/2r1/2(Vxy) -> is/3(ix,iy), Demux3/1  "Ixy"
  Demux2/2 -> [Iq]
  Demux3/1 -> [Ix]
  Demux1/6 -> 6s/2r1/6(W)
  Demux1/2 -> 6s/2r1/2(B)
  Demux1/5 -> 6s/2r1/5(V)
  Demux3/2 -> [Iy]
  Demux1/3 -> 6s/2r1/3(C)
  [TheI] -> Sin1/1, Sin/1, 6s/2r1/7(theta_e)
  Demux1/4 -> 6s/2r1/4(U)
  Demux1/1 -> 6s/2r1/1(A)
  6s/2r1/1(Vdq) -> is/2(id,iq), Demux2/1  "Idq"
  Mux/1 -> Demux1/1
  Sin/1 -> Mux1/1
  Sin1/1 -> Mux1/2
  Mux1/1 -> is/1(s,c)
  is/1(is_dq) -> Scope/1  "Is_dq"
  is/2(is_xy) -> Scope1/1  "Is_xy"

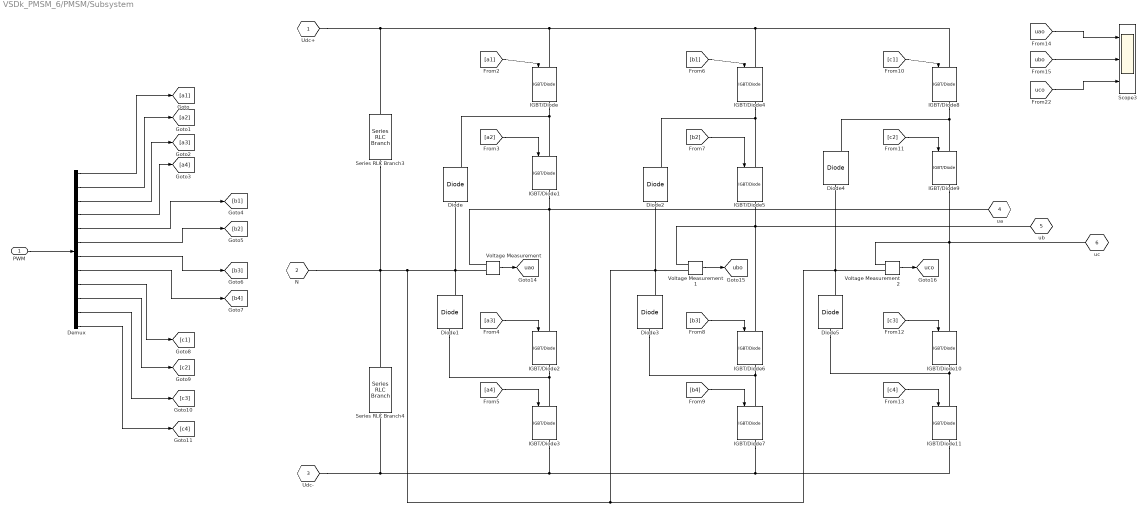
== system VSDk_PMSM_6/PMSM/Subsystem ==
  PWM : Inport
  Demux : Demux  Outputs=12
  Diode{,1..5} (6 alike) : spsDiodeLib/Diode  Ron=0.001  Lon=0  Vf=0.8  IC=0  UseSnubber=0  Rs=500  Cs=250e-9  Measurements=on
  IGBT/Diode{,1..11} (12 alike) : spsIGBTDiodeLib/IGBT//Diode  Ron=1e-3  Rs=1e5  Cs=inf  Measurements=on
  Scope3 : Scope  NumInputPorts=3
  Series RLC Branch3 : spsSeriesRLCBranchLib/Series RLC Branch  LConnTagsString=__new0  RConnTagsString=__new0  BranchType=RC  Resistance=0.01  Inductance=1e-3  SetiL0=off  InitialCurrent=0  Capacitance=670e-6  Setx0=off  InitialVoltage=0  Measurements=None
  Series RLC Branch4 : spsSeriesRLCBranchLib/Series RLC Branch  LConnTagsString=__new0  RConnTagsString=__new0  BranchType=RC  Resistance=0.01  Inductance=1e-3  SetiL0=off  InitialCurrent=0  Capacitance=670e-6  Setx0=off  InitialVoltage=0  Measurements=None
  Voltage Measurement : spsVoltageMeasurementLib/Voltage Measurement  PhasorSimulation=off  OutputType=Complex  PSBequivalent=0
  Voltage Measurement1 : spsVoltageMeasurementLib/Voltage Measurement  PhasorSimulation=off  OutputType=Complex  PSBequivalent=0
  Voltage Measurement2 : spsVoltageMeasurementLib/Voltage Measurement  PhasorSimulation=off  OutputType=Complex  PSBequivalent=0
  Udc+ : PMIOPort  Tag=PMCPort  Side=Left
  N : PMIOPort  Tag=PMCPort  Port=2  Side=Left
  Udc- : PMIOPort  Tag=PMCPort  Port=3  Side=Left
  ua : PMIOPort  Tag=PMCPort  Port=4  Side=Right
  ub : PMIOPort  Tag=PMCPort  Port=5  Side=Right
  uc : PMIOPort  Tag=PMCPort  Port=6  Side=Right
  tag scope: uao=global, ubo=global, uco=global
  wires:
  [c1] -> IGBT/Diode8/1
  [c3] -> IGBT/Diode10/1
  [c2] -> IGBT/Diode9/1
  [b3] -> IGBT/Diode6/1
  [a2] -> IGBT/Diode1/1
  [a1] -> IGBT/Diode/1
  [b1] -> IGBT/Diode4/1
  Voltage Measurement2/1 -> [uco]
  [b2] -> IGBT/Diode5/1
  [a4] -> IGBT/Diode3/1
  [c4] -> IGBT/Diode11/1
  Voltage Measurement/1 -> [uao]
  Voltage Measurement1/1 -> [ubo]
  [a3] -> IGBT/Diode2/1
  [b4] -> IGBT/Diode7/1
  PWM/1 -> Demux/1
  Demux/1 -> [a1]
  Demux/2 -> [a2]
  Demux/3 -> [a3]
  Demux/4 -> [a4]
  Demux/5 -> [b1]
  Demux/6 -> [b2]
  Demux/7 -> [b3]
  Demux/8 -> [b4]
  Demux/9 -> [c1]
  Demux/10 -> [c2]
  Demux/11 -> [c3]
  Demux/12 -> [c4]
  [uao] -> Scope3/1
  [uco] -> Scope3/3
  [ubo] -> Scope3/2
  connections:
  IGBT/Diode5/RConn1 -- Voltage Measurement1/LConn1 -- IGBT/Diode6/LConn1 -- ub/RConn1
  IGBT/Diode9/RConn1 -- Voltage Measurement2/LConn1 -- uc/RConn1 -- IGBT/Diode10/LConn1
  Series RLC Branch3/LConn1 -- Udc+/RConn1 -- IGBT/Diode4/LConn1 -- IGBT/Diode8/LConn1 -- IGBT/Diode/LConn1
  Series RLC Branch3/RConn1 -- N/RConn1 -- Series RLC Branch4/LConn1 -- Diode1/RConn1 -- Diode/LConn1 -- Voltage Measurement/LConn2 -- Diode3/RConn1 -- Diode2/LConn1 -- Voltage Measurement1/LConn2 -- Diode5/RConn1 -- Diode4/LConn1 -- Voltage Measurement2/LConn2
  Diode4/RConn1 -- IGBT/Diode9/LConn1 -- IGBT/Diode8/RConn1
  Diode1/LConn1 -- IGBT/Diode2/RConn1 -- IGBT/Diode3/LConn1
  IGBT/Diode1/RConn1 -- Voltage Measurement/LConn1 -- ua/RConn1 -- IGBT/Diode2/LConn1
  Diode/RConn1 -- IGBT/Diode/RConn1 -- IGBT/Diode1/LConn1
  Diode5/LConn1 -- IGBT/Diode10/RConn1 -- IGBT/Diode11/LConn1
  Series RLC Branch4/RConn1 -- Udc-/RConn1 -- IGBT/Diode7/RConn1 -- IGBT/Diode11/RConn1 -- IGBT/Diode3/RConn1
  Diode3/LConn1 -- IGBT/Diode6/RConn1 -- IGBT/Diode7/LConn1
  Diode2/RConn1 -- IGBT/Diode5/LConn1 -- IGBT/Diode4/RConn1

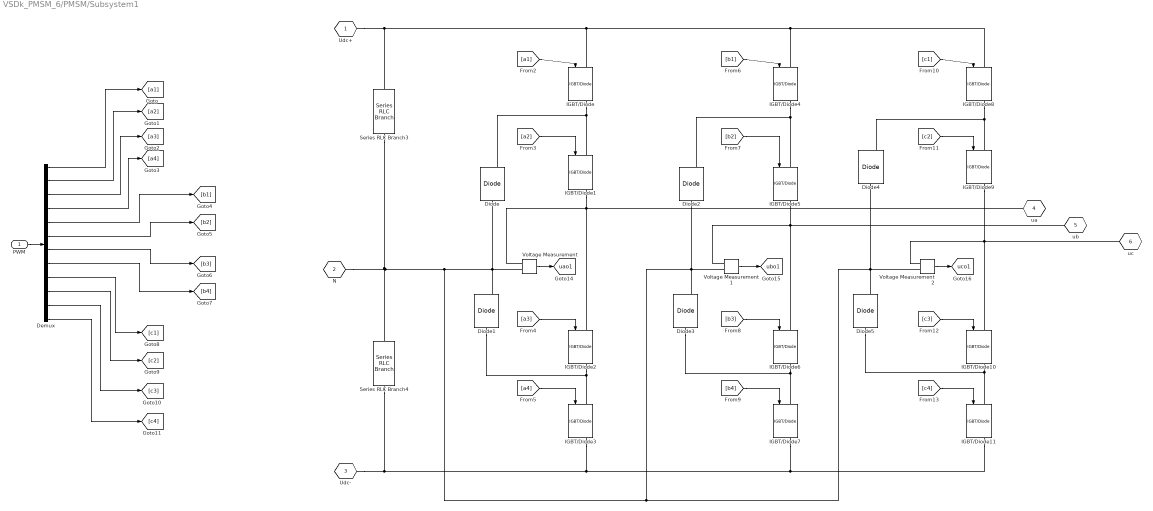
== system VSDk_PMSM_6/PMSM/Subsystem1 ==
  PWM : Inport
  Demux : Demux  Outputs=12
  Diode{,1..5} (6 alike) : spsDiodeLib/Diode  Ron=0.001  Lon=0  Vf=0.8  IC=0  UseSnubber=0  Rs=500  Cs=250e-9  Measurements=on
  IGBT/Diode{,1..11} (12 alike) : spsIGBTDiodeLib/IGBT//Diode  Ron=1e-3  Rs=1e5  Cs=inf  Measurements=on
  Series RLC Branch3 : spsSeriesRLCBranchLib/Series RLC Branch  LConnTagsString=__new0  RConnTagsString=__new0  BranchType=RC  Resistance=0.01  Inductance=1e-3  SetiL0=off  InitialCurrent=0  Capacitance=670e-6  Setx0=off  InitialVoltage=0  Measurements=None
  Series RLC Branch4 : spsSeriesRLCBranchLib/Series RLC Branch  LConnTagsString=__new0  RConnTagsString=__new0  BranchType=RC  Resistance=0.01  Inductance=1e-3  SetiL0=off  InitialCurrent=0  Capacitance=670e-6  Setx0=off  InitialVoltage=0  Measurements=None
  Voltage Measurement : spsVoltageMeasurementLib/Voltage Measurement  PhasorSimulation=off  OutputType=Complex  PSBequivalent=0
  Voltage Measurement1 : spsVoltageMeasurementLib/Voltage Measurement  PhasorSimulation=off  OutputType=Complex  PSBequivalent=0
  Voltage Measurement2 : spsVoltageMeasurementLib/Voltage Measurement  PhasorSimulation=off  OutputType=Complex  PSBequivalent=0
  Udc+ : PMIOPort  Tag=PMCPort  Side=Left
  N : PMIOPort  Tag=PMCPort  Port=2  Side=Left
  Udc- : PMIOPort  Tag=PMCPort  Port=3  Side=Left
  ua : PMIOPort  Tag=PMCPort  Port=4  Side=Right
  ub : PMIOPort  Tag=PMCPort  Port=5  Side=Right
  uc : PMIOPort  Tag=PMCPort  Port=6  Side=Right
  tag scope: uao1=global, ubo1=global, uco1=global
  wires:
  [c1] -> IGBT/Diode8/1
  [c3] -> IGBT/Diode10/1
  [c2] -> IGBT/Diode9/1
  [b3] -> IGBT/Diode6/1
  [a2] -> IGBT/Diode1/1
  [a1] -> IGBT/Diode/1
  [b1] -> IGBT/Diode4/1
  Voltage Measurement2/1 -> [uco1]
  [b2] -> IGBT/Diode5/1
  [a4] -> IGBT/Diode3/1
  [c4] -> IGBT/Diode11/1
  Voltage Measurement/1 -> [uao1]
  Voltage Measurement1/1 -> [ubo1]
  [a3] -> IGBT/Diode2/1
  [b4] -> IGBT/Diode7/1
  PWM/1 -> Demux/1
  Demux/1 -> [a1]
  Demux/2 -> [a2]
  Demux/3 -> [a3]
  Demux/4 -> [a4]
  Demux/5 -> [b1]
  Demux/6 -> [b2]
  Demux/7 -> [b3]
  Demux/8 -> [b4]
  Demux/9 -> [c1]
  Demux/10 -> [c2]
  Demux/11 -> [c3]
  Demux/12 -> [c4]
  connections:
  IGBT/Diode5/RConn1 -- Voltage Measurement1/LConn1 -- IGBT/Diode6/LConn1 -- ub/RConn1
  IGBT/Diode9/RConn1 -- Voltage Measurement2/LConn1 -- uc/RConn1 -- IGBT/Diode10/LConn1
  IGBT/Diode4/LConn1 -- IGBT/Diode8/LConn1 -- Udc+/RConn1 -- Series RLC Branch3/LConn1 -- IGBT/Diode/LConn1
  Series RLC Branch3/RConn1 -- Series RLC Branch4/LConn1 -- N/RConn1 -- Diode1/RConn1 -- Diode/LConn1 -- Voltage Measurement/LConn2 -- Diode3/RConn1 -- Diode2/LConn1 -- Voltage Measurement1/LConn2 -- Diode5/RConn1 -- Diode4/LConn1 -- Voltage Measurement2/LConn2
  Diode4/RConn1 -- IGBT/Diode9/LConn1 -- IGBT/Diode8/RConn1
  Diode1/LConn1 -- IGBT/Diode2/RConn1 -- IGBT/Diode3/LConn1
  IGBT/Diode1/RConn1 -- Voltage Measurement/LConn1 -- ua/RConn1 -- IGBT/Diode2/LConn1
  Diode/RConn1 -- IGBT/Diode/RConn1 -- IGBT/Diode1/LConn1
  Diode5/LConn1 -- IGBT/Diode10/RConn1 -- IGBT/Diode11/LConn1
  IGBT/Diode7/RConn1 -- IGBT/Diode11/RConn1 -- Udc-/RConn1 -- Series RLC Branch4/RConn1 -- IGBT/Diode3/RConn1
  Diode3/LConn1 -- IGBT/Diode6/RConn1 -- IGBT/Diode7/LConn1
  Diode2/RConn1 -- IGBT/Diode5/LConn1 -- IGBT/Diode4/RConn1

== system VSDk_PMSM_6/current regulator_Winding3/current regulator1 ==
  id_ref : Inport
  iq_ref : Inport  Port=2
  id_fdb : Inport  Port=3
  iq_fdb : Inport  Port=4
  Add5 : Sum  Inputs=+-
  Add8 : Sum  Inputs=+-
  Constant : Constant  Value=VDC
  MATLAB Function : MATLAB Function  TreatAsAtomicUnit=on
  PID Controller1 : slpidlib/PID Controller  Controller=PI  Form=Parallel  TimeDomain=Discrete-time  UseExternalTs=off  SampleTime=Ts  IntegratorMethod=Forward Euler  FilterMethod=Forward Euler  ControllerParametersSource=internal  P=Kp_iq_vsd  I=Ki_iq_vsd  UseKiTs=off  D=0  UseExternalDerivativeSource=off  N=100  UseFilter=on  TunerSelectOption=Transfer Function Based (PID Tuner App)  InitialConditionSource=internal  InitialConditionForIntegrator=0  InitialConditionForFilter=0  DifferentiatorICPrevScaledInput=0  ExternalReset=none  TrackingMode=off  Kt=1  LimitOutput=off  SatLimitsSource=internal  UpperSaturationLimit=inf  LowerSaturationLimit=-inf  LinearizeAsGain=on  AntiWindupMode=none  Kb=1  LimitIntegrator=off  UpperIntegratorSaturationLimit=inf  LowerIntegratorSaturationLimit=-inf  POutMin=[]  POutMax=[]  IOutMin=[]  IOutMax=[]  DOutMin=[]  DOutMax=[]  NOutMin=[]  NOutMax=[]  SumOutMin=[]  SumOutMax=[]  SaturationOutMin=[]  SaturationOutMax=[]  PParamMin=[]  PParamMax=[]  IParamMin=[]  IParamMax=[]  DParamMin=[]  DParamMax=[]  NParamMin=[]  NParamMax=[]  KbParamMin=[]  KbParamMax=[]  KtParamMin=[]  KtParamMax=[]  KbOutMin=[]  KbOutMax=[]  KtOutMin=[]  KtOutMax=[]  IntegratorOutMin=[]  IntegratorOutMax=[]  FilterOutMin=[]  FilterOutMax=[]  SumI1OutMin=[]  SumI1OutMax=[]  SumI2OutMin=[]  SumI2OutMax=[]  SumI3OutMin=[]  SumI3OutMax=[]  SumI4OutMin=[]  SumI4OutMax=[]  SumDOutMin=[]  SumDOutMax=[]  DifferentiatorOutMin=[]  DifferentiatorOutMax=[]  FilterDiffOutCoefMin=[]  FilterDiffOutCoefMax=[]  ReciprocalOutMin=[]  ReciprocalOutMax=[]  SumDenOutMin=[]  SumDenOutMax=[]  SumNumOutMin=[]  SumNumOutMax=[]  DivideOutMin=[]  DivideOutMax=[]  UdiffTsProdOutMin=[]  UdiffTsProdOutMax=[]  NTsProdOutMin=[]  NTsProdOutMax=[]  UintegralTsProdOutMin=[]  UintegralTsProdOutMax=[]  UngainTsProdOutMin=[]  UngainTsProdOutMax=[]  ClampingZeroOutDataTypeStr=Inherit: Inherit via back propagation  ClampingZeroOutMin=[]  ClampingZeroOutMax=[]  FilterDenConstantOutDataTypeStr=Inherit: Inherit via back propagation  FilterDenConstantOutMin=[]  FilterDenConstantOutMax=[]  PCopyOutDataTypeStr=Inherit: Inherit via back propagation  PCopyOutMin=[]  PCopyOutMax=[]  NCopyOutDataTypeStr=Inherit: Inherit via back propagation  NCopyOutMin=[]  NCopyOutMax=[]  IntegratorContinuousStateAttributes=''  IntegratorStateMustResolveToSignalObject=off  IntegratorRTWStateStorageClass=Auto  FilterContinuousStateAttributes=''  FilterStateMustResolveToSignalObject=off  FilterRTWStateStorageClass=Auto  ParallelPVariant=InternalParameters  IdealPVariant=Disabled  IVariant=InternalParameters  DVariant=Disabled  IntegratorVariant=Discrete  SatVariant=Disabled  AWVariant=Passthrough  PCopyVariant=Disabled  TRVariant=Disabled  FdbkBlocksVariant=Forward  IdealPFdbkVariant=Disabled  SatFdbkVariant=Disabled  DerivativeFilterVariant=Disabled  NVariant=Disabled  NCopyVariant=Disabled_SignalSpec  FilterICVariant=Disabled  IntegratorICVariant=InternalICs  ExternalResetVariant=Disabled  TRSumVariant=Passthrough  SumFdbkVariant=Disabled  SumVariant=Sum_PI  TsampFilterVariant=InternalTs  TsampNgainVariant=Passthrough  TsampIntegralVariant=Disabled_SignalSpec  ExternalSaturationOutDataTypeStr=Inherit: Same as second input  DerivativeSourceVariant=Disabled
  PID Controller2 : slpidlib/PID Controller  Controller=PI  Form=Parallel  TimeDomain=Discrete-time  UseExternalTs=off  SampleTime=Ts  IntegratorMethod=Forward Euler  FilterMethod=Forward Euler  ControllerParametersSource=internal  P=Kp_id_vsd  I=Ki_id_vsd  UseKiTs=off  D=0  UseExternalDerivativeSource=off  N=100  UseFilter=on  TunerSelectOption=Transfer Function Based (PID Tuner App)  InitialConditionSource=internal  InitialConditionForIntegrator=0  InitialConditionForFilter=0  DifferentiatorICPrevScaledInput=0  ExternalReset=none  TrackingMode=off  Kt=1  LimitOutput=off  SatLimitsSource=internal  UpperSaturationLimit=inf  LowerSaturationLimit=-inf  LinearizeAsGain=on  AntiWindupMode=none  Kb=1  LimitIntegrator=off  UpperIntegratorSaturationLimit=inf  LowerIntegratorSaturationLimit=-inf  POutMin=[]  POutMax=[]  IOutMin=[]  IOutMax=[]  DOutMin=[]  DOutMax=[]  NOutMin=[]  NOutMax=[]  SumOutMin=[]  SumOutMax=[]  SaturationOutMin=[]  SaturationOutMax=[]  PParamMin=[]  PParamMax=[]  IParamMin=[]  IParamMax=[]  DParamMin=[]  DParamMax=[]  NParamMin=[]  NParamMax=[]  KbParamMin=[]  KbParamMax=[]  KtParamMin=[]  KtParamMax=[]  KbOutMin=[]  KbOutMax=[]  KtOutMin=[]  KtOutMax=[]  IntegratorOutMin=[]  IntegratorOutMax=[]  FilterOutMin=[]  FilterOutMax=[]  SumI1OutMin=[]  SumI1OutMax=[]  SumI2OutMin=[]  SumI2OutMax=[]  SumI3OutMin=[]  SumI3OutMax=[]  SumI4OutMin=[]  SumI4OutMax=[]  SumDOutMin=[]  SumDOutMax=[]  DifferentiatorOutMin=[]  DifferentiatorOutMax=[]  FilterDiffOutCoefMin=[]  FilterDiffOutCoefMax=[]  ReciprocalOutMin=[]  ReciprocalOutMax=[]  SumDenOutMin=[]  SumDenOutMax=[]  SumNumOutMin=[]  SumNumOutMax=[]  DivideOutMin=[]  DivideOutMax=[]  UdiffTsProdOutMin=[]  UdiffTsProdOutMax=[]  NTsProdOutMin=[]  NTsProdOutMax=[]  UintegralTsProdOutMin=[]  UintegralTsProdOutMax=[]  UngainTsProdOutMin=[]  UngainTsProdOutMax=[]  ClampingZeroOutDataTypeStr=Inherit: Inherit via back propagation  ClampingZeroOutMin=[]  ClampingZeroOutMax=[]  FilterDenConstantOutDataTypeStr=Inherit: Inherit via back propagation  FilterDenConstantOutMin=[]  FilterDenConstantOutMax=[]  PCopyOutDataTypeStr=Inherit: Inherit via back propagation  PCopyOutMin=[]  PCopyOutMax=[]  NCopyOutDataTypeStr=Inherit: Inherit via back propagation  NCopyOutMin=[]  NCopyOutMax=[]  IntegratorContinuousStateAttributes=''  IntegratorStateMustResolveToSignalObject=off  IntegratorRTWStateStorageClass=Auto  FilterContinuousStateAttributes=''  FilterStateMustResolveToSignalObject=off  FilterRTWStateStorageClass=Auto  ParallelPVariant=InternalParameters  IdealPVariant=Disabled  IVariant=InternalParameters  DVariant=Disabled  IntegratorVariant=Discrete  SatVariant=Disabled  AWVariant=Passthrough  PCopyVariant=Disabled  TRVariant=Disabled  FdbkBlocksVariant=Forward  IdealPFdbkVariant=Disabled  SatFdbkVariant=Disabled  DerivativeFilterVariant=Disabled  NVariant=Disabled  NCopyVariant=Disabled_SignalSpec  FilterICVariant=Disabled  IntegratorICVariant=InternalICs  ExternalResetVariant=Disabled  TRSumVariant=Passthrough  SumFdbkVariant=Disabled  SumVariant=Sum_PI  TsampFilterVariant=InternalTs  TsampNgainVariant=Passthrough  TsampIntegralVariant=Disabled_SignalSpec  ExternalSaturationOutDataTypeStr=Inherit: Same as second input  DerivativeSourceVariant=Disabled
  Scope : Scope  NumInputPorts=2
  Scope1 : Scope  NumInputPorts=2
  Mq : Outport
  Md : Outport  Port=2
  wires:
  Constant/1 -> MATLAB Function/3(VDC)
  MATLAB Function/2(ud) -> Scope1/2, Md/1
  MATLAB Function/1(uq) -> Scope1/1, Mq/1
  PID Controller2/1 -> Scope/2, MATLAB Function/2(ud_in)
  PID Controller1/1 -> Scope/1, MATLAB Function/1(uq_in)
  id_ref/1 -> Add8/1
  id_fdb/1 -> Add8/2
  iq_ref/1 -> Add5/1
  iq_fdb/1 -> Add5/2
  Add5/1 -> PID Controller1/1
  Add8/1 -> PID Controller2/1
